simulink model "Kalman_Filter"  (R2025b)
settings: Solver=VariableStepAuto  StartTime=0.0  StopTime=10.0  RelTol=1e-3
undefined symbols (not defined in the file): A, b, B, c, C, Continuous, g, I, kb, kt, l, M, m, r, Rm, Time
libraries: vrlib x3, simulink x2, ctrlSharedLib x1
settings Model: Creator=Usuario  LastModifiedBy=joelalfaro

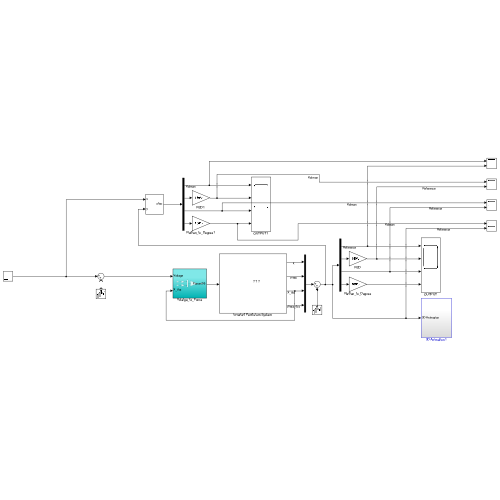
[thumbnail: Simulink's stored preview of the top-level diagram]
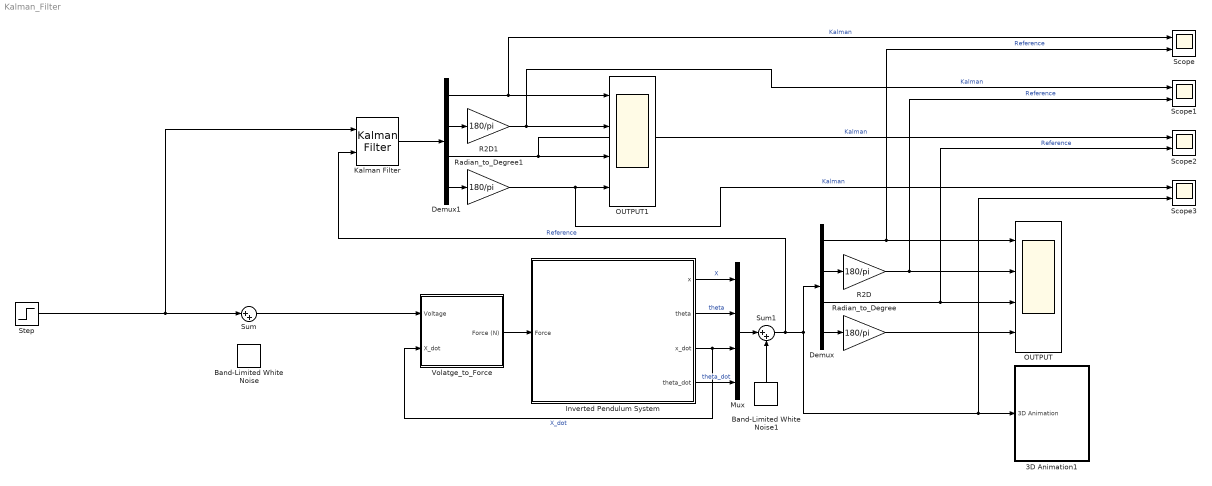
== system Kalman_Filter ==
  3D Animation1 : Subsystem
  Band-Limited White Noise : simulink/Sources/Band-Limited White Noise  Cov=[0.000015]  Ts=0.1  seed=[23341]
  Band-Limited White Noise1 : simulink/Sources/Band-Limited White Noise  Cov=[0.00015]  Ts=0.1  seed=[23341]
  Demux : Demux
  Demux1 : Demux
  Inverted Pendulum System : Subsystem
      mask Display: image('ip_model.png');
  Kalman Filter : ctrlSharedLib/Kalman Filter  TimeDomain=Continuous-Time  UseCurrentEstimator=on  ModelSource=Individual A, B, C, D matrices  ModelSourceVariable=ss(0.95,1,1,0,1)  A=A  B=B  C=C  D=[0;0;0;0]  NumberOfStates=1  NumberOfInputs=1  NumberOfOutputs=1  InitialEstimateSource=Dialog  X0=0  P0=10  UseK=off  UseGH=off  NumberOfProcessNoiseInputs=1  G=1  TimeInvariantG=on  H=0  TimeInvariantH=on  Q=diag([0 0 0 0.0001])  TimeInvariantQ=on  R=0.005  TimeInvariantR=on  N=0  TimeInvariantN=on  AddInputPort=on  AddEnablePort=off  OutputEstimatedY=off  OutputP=off  Ts=-1
  Mux : Mux
  OUTPUT : Scope  NumInputPorts=4
      settings: ActiveDisplayYMinimum=-0.3923621314060084  ActiveDisplayYMaximum=5.0103932741714461  YLabel=X (m)  DataLoggingVariableName=ScopeData4
  OUTPUT1 : Scope  NumInputPorts=4
      settings: ActiveDisplayYMinimum=-0.6191677485074718  ActiveDisplayYMaximum=4.7220611123421641  YLabel=X (m)
  R2D : Gain  Gain=180/pi
  R2D1 : Gain  Gain=180/pi
  Radian_to_Degree : Gain  Gain=180/pi
  Radian_to_Degree1 : Gain  Gain=180/pi
  Scope{,1..3} (4 alike) : Scope  NumInputPorts=2
      Scope settings: ActiveDisplayYMinimum=-0.65439109943298335  ActiveDisplayYMaximum=5.0395076039522211
      Scope1 settings: ActiveDisplayYMinimum=-194.56146995307557  ActiveDisplayYMaximum=200.2747574357376  DataLoggingVariableName=ScopeData2
      Scope2 settings: ActiveDisplayYMinimum=-0.761515400372417  ActiveDisplayYMaximum=0.96358403387624769  DataLoggingVariableName=ScopeData3
      Scope3 settings: ActiveDisplayYMinimum=-1300.2189091732523  ActiveDisplayYMaximum=974.22475065068465  DataLoggingVariableName=ScopeData5
  Step : Step  After=pi  SampleTime=0
  Sum : Sum  Inputs=|++
  Sum1 : Sum  Inputs=|++
  Volatge_to_Force : Subsystem
  wires:
  Demux/4 -> Radian_to_Degree/1
  Demux/2 -> R2D/1
  Demux/3 -> Scope2/2, OUTPUT/3  "Reference"
  Inverted Pendulum System/1(x) -> Mux/1  "X"
  R2D/1 -> Scope1/2, OUTPUT/2  "Reference"
  Radian_to_Degree/1 -> OUTPUT/4
  Volatge_to_Force/1(Force (N)) -> Inverted Pendulum System/1(Force)
  Inverted Pendulum System/4(theta_dot) -> Mux/4  "theta_dot"
  Inverted Pendulum System/2(theta) -> Mux/2  "theta"
  Inverted Pendulum System/3(x_dot) -> Volatge_to_Force/2(X_dot), Mux/3  "X_dot"
  Demux1/1 -> Scope/1, OUTPUT1/1  "Kalman"
  Demux1/2 -> R2D1/1
  Demux1/3 -> Scope2/1, OUTPUT1/3  "Kalman"
  R2D1/1 -> Scope1/1, OUTPUT1/2  "Kalman"
  Demux1/4 -> Radian_to_Degree1/1
  Radian_to_Degree1/1 -> Scope3/1, OUTPUT1/4  "Kalman"
  Mux/1 -> Sum1/1
  Band-Limited White Noise1/1 -> Sum1/2
  Sum1/1 -> Kalman Filter/2, Demux/1, Scope3/2, 3D Animation1/1(3D Animation)  "Reference"
  Step/1 -> Sum/1, Kalman Filter/1
  Sum/1 -> Volatge_to_Force/1(Voltage)
  Kalman Filter/1 -> Demux1/1
  Demux/1 -> Scope/2, OUTPUT/1  "Reference"

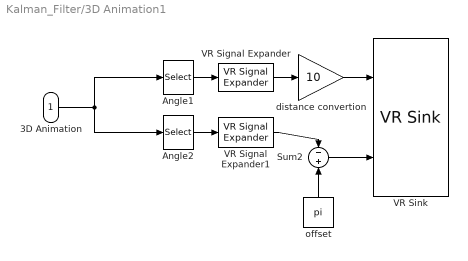
== system Kalman_Filter/3D Animation1 ==
  3D Animation : Inport
  Angle1 : Selector  InputPortWidth=4  IndexOptions=Index vector (dialog)  Indices=[1]  OutputSizes=1
  Angle2 : Selector  InputPortWidth=4  IndexOptions=Index vector (dialog)  Indices=[2]  OutputSizes=1
  Sum2 : Sum  Inputs=-|+
  VR Signal Expander : vrlib/VR Signal Expander  outwidth=3  outidx=[1]
  VR Signal Expander1 : vrlib/VR Signal Expander  outwidth=4  outidx=[4]
  VR Sink : vrlib/VR Sink  InstantiateOnLoad=on  SampleTime=0.02  ViewEnable=on  RemoteChange=off  RemoteView=off  FieldsWritten=cart.translation.3.1.1.double#joint.rotation.4.1.1.double  WorldFileName=Inverted_pendulum12.wrl  AutoView=off  VideoDimensions=[]  AllowVariableSize=off
  distance convertion : Gain  Gain=10
  offset : Constant  Value=pi
  wires:
  VR Signal Expander/1 -> distance convertion/1
  3D Animation/1 -> Angle2/1, Angle1/1
  Angle1/1 -> VR Signal Expander/1
  Angle2/1 -> VR Signal Expander1/1
  offset/1 -> Sum2/2
  Sum2/1 -> VR Sink/2
  VR Signal Expander1/1 -> Sum2/1
  distance convertion/1 -> VR Sink/1

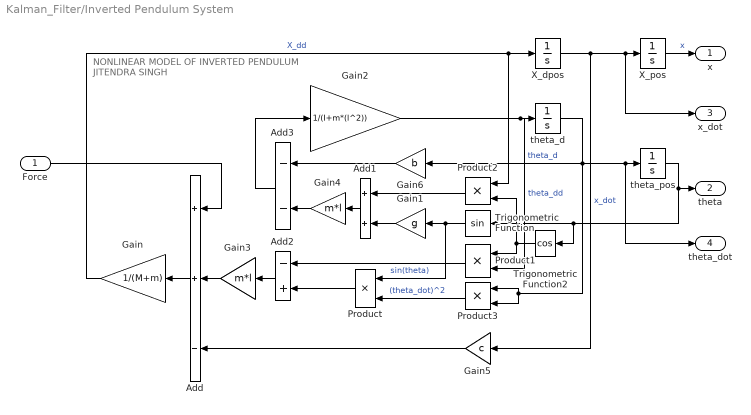
== system Kalman_Filter/Inverted Pendulum System ==
  note: NONLINEAR MODEL OF
      | INVERTED PENDULUM
      | JITENDRA SINGH
  Force : Inport
  Add : Sum  Inputs=++-
  Add1 : Sum
  Add2 : Sum  Inputs=-+
  Add3 : Sum  Inputs=--
  Gain : Gain  Gain=1/(M+m)
  Gain1 : Gain  Gain=g
  Gain2 : Gain  Gain=1/(I+m*(l^2))
  Gain3 : Gain  Gain=m*l
  Gain4 : Gain  Gain=m*l
  Gain5 : Gain  Gain=c
  Gain6 : Gain  Gain=b
  Product{,1..3} (4 alike) : Product
  Trigonometric Function : Trigonometry
  Trigonometric Function2 : Trigonometry  Operator=cos
  X_dpos : Integrator
  X_pos : Integrator  InitialCondition=0.2
  theta_d : Integrator
  theta_pos : Integrator  InitialCondition=160*(pi/180)
  x : Outport  VectorParamsAs1DForOutWhenUnconnected=off
  theta : Outport  Port=2  VectorParamsAs1DForOutWhenUnconnected=off
  x_dot : Outport  Port=3  VectorParamsAs1DForOutWhenUnconnected=off
  theta_dot : Outport  Port=4  VectorParamsAs1DForOutWhenUnconnected=off
  wires:
  Gain5/1 -> Add/3
  Add2/1 -> Gain3/1
  Add3/1 -> Gain2/1
  Trigonometric Function2/1 -> Product2/2, Product1/1
  Trigonometric Function/1 -> Product/1, Gain1/1  "sin(theta)"
  Gain3/1 -> Add/2
  theta_d/1 -> Product3/2, Product3/1, Gain6/1, theta_dot/1, theta_pos/1  "theta_d"
  Product2/1 -> Add1/1
  Product/1 -> Add2/2
  Gain4/1 -> Add3/2
  Product3/1 -> Product/2  "(theta_dot)^2"
  X_pos/1 -> x/1  "x"
  Product1/1 -> Add2/1
  Gain/1 -> X_dpos/1, Product2/1  "X_dd"
  Add/1 -> Gain/1
  Gain2/1 -> Product1/2, theta_d/1  "theta_dd"
  Gain6/1 -> Add3/1
  theta_pos/1 -> Trigonometric Function2/1, Trigonometric Function/1, theta/1
  Force/1 -> Add/1
  Gain1/1 -> Add1/2
  X_dpos/1 -> x_dot/1, X_pos/1, Gain5/1  "x_dot"
  Add1/1 -> Gain4/1

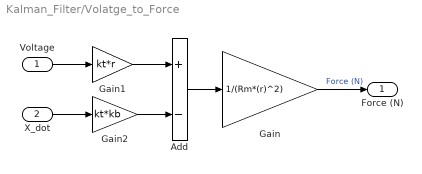
== system Kalman_Filter/Volatge_to_Force ==
  Voltage : Inport
  X_dot : Inport  Port=2
  Add : Sum  Inputs=+-
  Gain : Gain  Gain=1/(Rm*(r)^2)
  Gain1 : Gain  Gain=kt*r
  Gain2 : Gain  Gain=kt*kb
  Force (N) : Outport  VectorParamsAs1DForOutWhenUnconnected=off
  wires:
  Gain1/1 -> Add/1
  Gain2/1 -> Add/2
  Voltage/1 -> Gain1/1
  Gain/1 -> Force (N)/1  "Force (N)"
  X_dot/1 -> Gain2/1
  Add/1 -> Gain/1
